simulink model "m01"  (R2025a)
settings: Solver=FixedStepAuto  StartTime=0.0  StopTime=20  FixedStep=dtsim  MaxStep=1e-3  RelTol=1e-3
values from neighbouring files (symbols this model uses):
  mp = block.DialogPrm(2).Data    [m01_anim.m]    (also in m01_params.m = [])
settings Model: Creator=hgeyer  LastModifiedBy=hgeyer

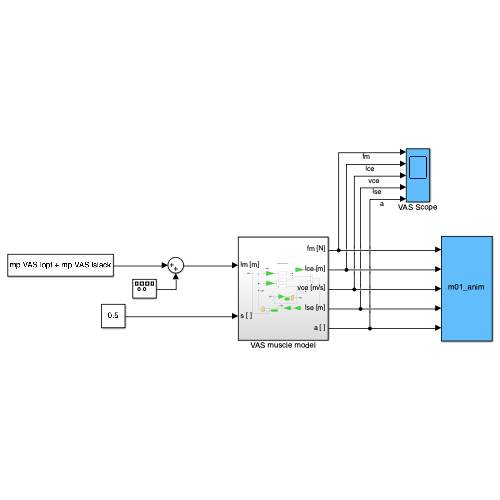
[thumbnail: Simulink's stored preview of the top-level diagram]
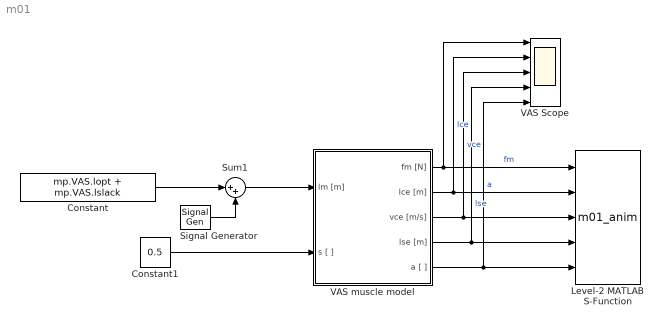
== system m01 ==
  Constant : Constant  Value=mp.VAS.lopt + mp.VAS.lslack
  Constant1 : Constant  Value=0.5
  Level-2 MATLAB S-Function : M-S-Function  FunctionName=m01_anim  Parameters=rtf_anim, mp
  Signal Generator : SignalGenerator  Amplitude=0.3 * mp.VAS.lopt  Frequency=0.5
  Sum1 : Sum  Inputs=|++
  VAS Scope : Scope  NumInputPorts=5
      settings: ActiveDisplayYMinimum=-526.76194095868971  ActiveDisplayYMaximum=4740.8574686282082
  VAS muscle model : Subsystem
  wires:
  VAS muscle model/1(fm [N]) -> VAS Scope/1, Level-2 MATLAB S-Function/1  "fm"
  VAS muscle model/2(lce [m]) -> VAS Scope/2, Level-2 MATLAB S-Function/2  "lce"
  VAS muscle model/3(vce [m/s]) -> VAS Scope/3, Level-2 MATLAB S-Function/3  "vce"
  VAS muscle model/4(lse [m]) -> VAS Scope/4, Level-2 MATLAB S-Function/4  "lse"
  VAS muscle model/5(a [ ]) -> VAS Scope/5, Level-2 MATLAB S-Function/5  "a"
  Constant1/1 -> VAS muscle model/2(s [ ])
  Constant/1 -> Sum1/1
  Sum1/1 -> VAS muscle model/1(lm [m])
  Signal Generator/1 -> Sum1/2

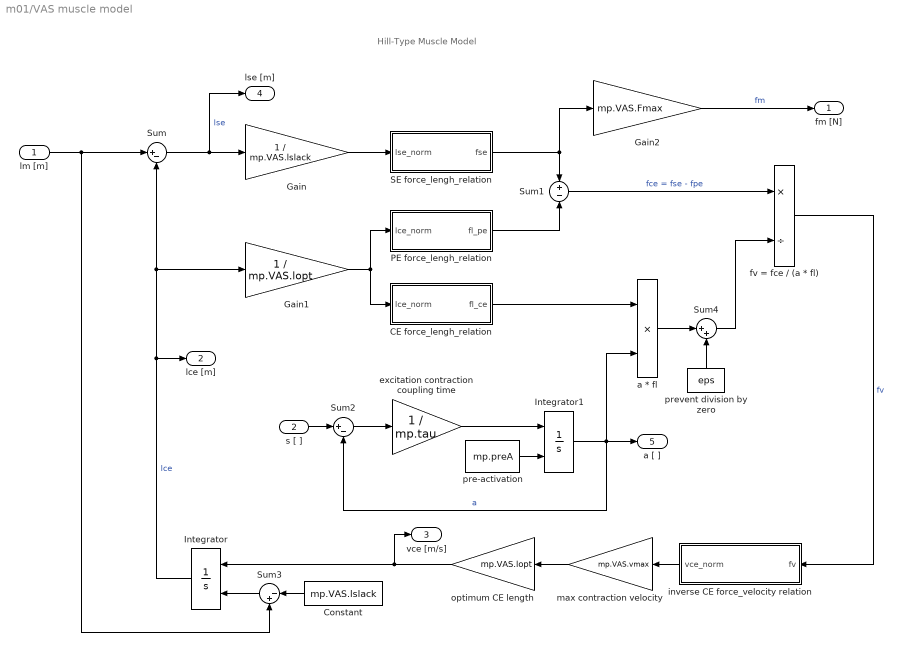
== system m01/VAS muscle model ==
  note: Hill-Type Muscle Model
  lm [m] : Inport
  s [ ] : Inport  Port=2
  CE force_lengh_relation : MATLAB Function  TreatAsAtomicUnit=on
  Constant : Constant  Value=mp.VAS.lslack
  Gain : Gain  Gain=1 / mp.VAS.lslack
  Gain1 : Gain  Gain=1 / mp.VAS.lopt
  Gain2 : Gain  Gain=mp.VAS.Fmax
  Integrator : Integrator  InitialConditionSource=external
  Integrator1 : Integrator  InitialConditionSource=external
  PE force_lengh_relation : MATLAB Function  TreatAsAtomicUnit=on
  SE force_lengh_relation : MATLAB Function  TreatAsAtomicUnit=on
  Sum : Sum  Inputs=|+-
  Sum1 : Sum  Inputs=+-
  Sum2 : Sum  Inputs=|+-
  Sum3 : Sum  Inputs=|-+
  Sum4 : Sum  Inputs=|++
  a * fl : Product  Inputs=**
  excitation contraction coupling time : Gain  Gain=1 / mp.tau
  fv = fce / (a * fl) : Product  Inputs=*/
  inverse CE force_velocity relation : MATLAB Function  TreatAsAtomicUnit=on
  max contraction velocity : Gain  Gain=mp.VAS.vmax
  optimum CE length : Gain  Gain=mp.VAS.lopt
  pre-activation : Constant  Value=mp.preA
  prevent division by zero : Constant  Value=eps
  fm [N] : Outport
  lce [m] : Outport  Port=2
  vce [m/s] : Outport  Port=3
  lse [m] : Outport  Port=4
  a [ ] : Outport  Port=5
  wires:
  Gain2/1 -> fm [N]/1  "fm"
  optimum CE length/1 -> vce [m/s]/1, Integrator/1
  a * fl/1 -> Sum4/1
  Sum2/1 -> excitation contraction coupling time/1
  Gain/1 -> SE force_lengh_relation/1(lse_norm)
  s [ ]/1 -> Sum2/1
  fv = fce / (a * fl)/1 -> inverse CE force_velocity relation/1(fv)  "fv"
  inverse CE force_velocity relation/1(vce_norm) -> max contraction velocity/1
  Sum/1 -> lse [m]/1, Gain/1  "lse"
  Integrator/1 -> lce [m]/1, Gain1/1, Sum/2  "lce"
  SE force_lengh_relation/1(fse) -> Gain2/1, Sum1/1
  PE force_lengh_relation/1(fl_pe) -> Sum1/2
  max contraction velocity/1 -> optimum CE length/1
  Sum3/1 -> Integrator/2
  pre-activation/1 -> Integrator1/2
  CE force_lengh_relation/1(fl_ce) -> a * fl/1
  lm [m]/1 -> Sum3/2, Sum/1
  Sum4/1 -> fv = fce / (a * fl)/2
  Constant/1 -> Sum3/1
  prevent division by zero/1 -> Sum4/2
  excitation contraction coupling time/1 -> Integrator1/1
  Gain1/1 -> CE force_lengh_relation/1(lce_norm), PE force_lengh_relation/1(lce_norm)
  Integrator1/1 -> a [ ]/1, Sum2/2, a * fl/2  "a"
  Sum1/1 -> fv = fce / (a * fl)/1  "fce = fse - fpe"

== matlab function m01/VAS muscle model/SE force_lengh_relation ==
  data: lse_norm input; fse output; mp parameter
function fse = fcn(lse_norm, mp)
% wraps force length relation of series elasticity

fse = SE_force_length_relation(lse_norm, mp);

== matlab function m01/VAS muscle model/PE force_lengh_relation ==
  data: lce_norm input; fl_pe output; mp parameter
function fl_pe = fcn(lce_norm, mp)
% wraps force length relation of parallel elasticity

fl_pe = PE_force_length_relation(lce_norm, mp);

== matlab function m01/VAS muscle model/inverse CE force_velocity relation ==
  data: fv input; vce_norm output; mp parameter
function vce_norm = fcn(fv, mp)
% wraps inverse force velocity relation of contractile element

vce_norm = CE_inverse_force_velocity_relation(fv, mp);

== matlab function m01/VAS muscle model/CE force_lengh_relation ==
  data: lce_norm input; fl_ce output; mp parameter
function fl_ce = fcn(lce_norm, mp)
% wraps force length relation of contractile element

fl_ce = CE_force_length_relation(lce_norm, mp);
